simulink model "W07_alloc_chain"  (R2024b)
settings: Solver=ode4  StartTime=0  StopTime=T_final  FixedStep=h  RelTol=1e-3
InitFcn:
  | addpath(fullfile(fileparts(fileparts(fileparts(get_param(bdroot, 'FileName')))), '_tools'), fileparts(get_param(bdroot, 'FileName'))); run_alone('W07', bdroot);
StopFcn:
  | W07_plot_ca;
values from neighbouring files (symbols this model uses):
  alpha_lim = cfg.alpha_max(1)    [W07_0_setup.m]
  B_alloc = cfg.B    [W07_0_setup.m]
  beta_c = pi/2    (= 1.57079632679)    [W07_0_setup.m]
  eps_reg = 1e-4    (= 0.0001)    [W07_0_setup.m]    (also in W07_alloc_run.m)
  k_neg = cfg.k_neg    [W07_0_setup.m]
  k_pos = cfg.k_pos    [W07_0_setup.m]
  law = 4    [W07_0_setup.m]
  mp = 25    [W07_0_setup.m]
  n_max = cfg.n_max    [W07_0_setup.m]    (also in W07_plot_ca.m = base_num('n_max',      103.93); W07_plot_sat.m = base_var('n_max',      103.931))
  n_min = cfg.n_min    [W07_0_setup.m]    (also in W07_plot_ca.m = base_num('n_min',     -101.74); W07_plot_sat.m = base_var('n_min',     -101.737))
  Q_tau = eye(3)    [W07_0_setup.m]    (also in W07_alloc_run.m)
  quad = [cfg.pos ; cfg.alpha_max ; cfg.mount]    [W07_0_setup.m]
  rp = [0.05 0 -0.35]'    [W07_0_setup.m]
  T_neg = cfg.k_neg * cfg.n_min^2    [W07_0_setup.m]    (also in W07_plot_ca.m = base_num('T_neg',       66.708); W07_plot_sat.m = base_var('T_neg',        66.708))
  T_pos = cfg.k_pos * cfg.n_max^2    [W07_0_setup.m]    (also in W07_plot_ca.m = base_num('T_pos',      119.682); W07_plot_sat.m = base_var('T_pos',       119.682))
  tau_cmd = [0; 40; 0]    [W07_0_setup.m]
  V_c = 0.0    (= 0)    [W07_0_setup.m]
  W_alloc = diag(repmat([1 10], 1, 4))    [W07_0_setup.m]
  x0 = zeros(12,1)    [W07_0_setup.m]
settings Model: Creator=admin  LastModifiedBy=admin
settings DataIOCC: ReturnWorkspaceOutputs=off

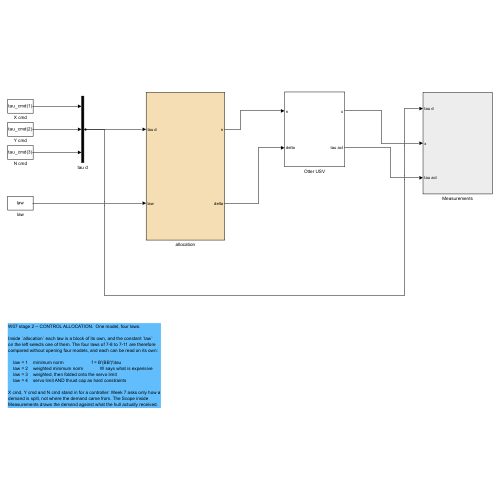
[thumbnail: Simulink's stored preview of the top-level diagram]
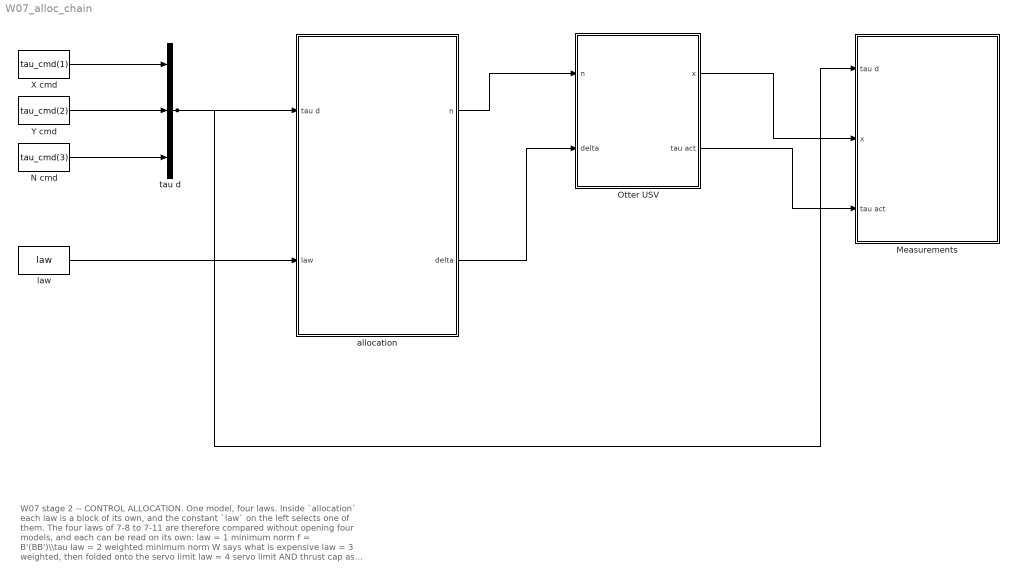
== system W07_alloc_chain ==
  note: W07 stage 2 -- CONTROL ALLOCATION.  One model, four laws.
      |
      | Inside `allocation` each law is a block of its own, and the constant `law`
      | on the left selects one of them. The four laws of 7-8 to 7-11 are therefore
      | compared without opening four models, and each can be read on its own:
      |
      |     law = 1    minimum norm                      f = B'(BB')\\tau
      |     law = 2    weighted minimum norm             W says what is expensive
      |     law = 3    weighted, then folded onto the servo limit
      |     law = 4    servo limit AND thrust cap as hard constraints
      |
      | X cmd, Y cmd and N cmd stand in for a controller: Week 7 asks only how a
      | demand is split, not where the demand came from. The Scope inside
      | Measurements draws the demand against what the hull actually received.
  Measurements : Subsystem
  N cmd : Constant  Value=tau_cmd(3)
  Otter USV : Subsystem
  X cmd : Constant  Value=tau_cmd(1)
  Y cmd : Constant  Value=tau_cmd(2)
  allocation : Subsystem
  law : Constant  Value=law
  tau d : Mux  Inputs=3
  wires:
  tau d/1 -> allocation/1(tau d), Measurements/1(tau d)
  law/1 -> allocation/2(law)
  X cmd/1 -> tau d/1
  Y cmd/1 -> tau d/2
  N cmd/1 -> tau d/3
  allocation/1(n) -> Otter USV/1(n)
  allocation/2(delta) -> Otter USV/2(delta)
  Otter USV/1(x) -> Measurements/2(x)
  Otter USV/2(tau act) -> Measurements/3(tau act)

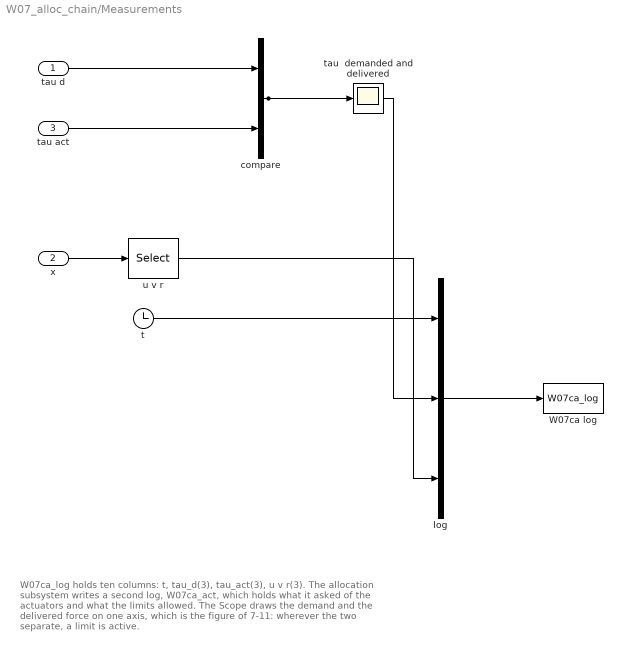
== system W07_alloc_chain/Measurements ==
  note: W07ca_log holds ten columns:  t,  tau_d(3),  tau_act(3),  u v r(3).
      | The allocation subsystem writes a second log, W07ca_act, which holds what
      | it asked of the actuators and what the limits allowed.
      |
      | The Scope draws the demand and the delivered force on one axis, which is
      | the figure of 7-11: wherever the two separate, a limit is active.
  tau d : Inport
  x : Inport  Port=2
  tau act : Inport  Port=3
  W07ca log : ToWorkspace  VariableName=W07ca_log  SampleTime=-1
  compare : Mux  Inputs=2
  log : Mux  Inputs=3
  t : Clock
  tau  demanded and delivered : Scope
  u v r : Selector  InputPortWidth=12  IndexOptions=Index vector (dialog)  Indices=[1 2 3]  OutputSizes=1
  wires:
  tau d/1 -> compare/1
  tau act/1 -> compare/2
  x/1 -> u v r/1
  t/1 -> log/1
  compare/1 -> tau  demanded and delivered/1, log/2
  log/1 -> W07ca log/1
  u v r/1 -> log/3

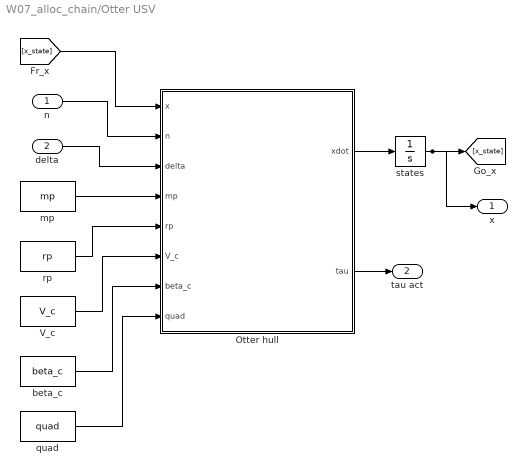
== system W07_alloc_chain/Otter USV ==
  n : Inport
  delta : Inport  Port=2
  Otter hull : MATLAB Function  TreatAsAtomicUnit=on
  V_c : Constant  Value=V_c
  beta_c : Constant  Value=beta_c
  mp : Constant  Value=mp
  quad : Constant  Value=quad
  rp : Constant  Value=rp
  states : Integrator  InitialCondition=x0
  x : Outport
  tau act : Outport  Port=2
  wires:
  rp/1 -> Otter hull/5(rp)
  delta/1 -> Otter hull/3(delta)
  [x_state] -> Otter hull/1(x)
  beta_c/1 -> Otter hull/7(beta_c)
  V_c/1 -> Otter hull/6(V_c)
  n/1 -> Otter hull/2(n)
  mp/1 -> Otter hull/4(mp)
  quad/1 -> Otter hull/8(quad)
  Otter hull/1(xdot) -> states/1
  states/1 -> [x_state], x/1
  Otter hull/2(tau) -> tau act/1

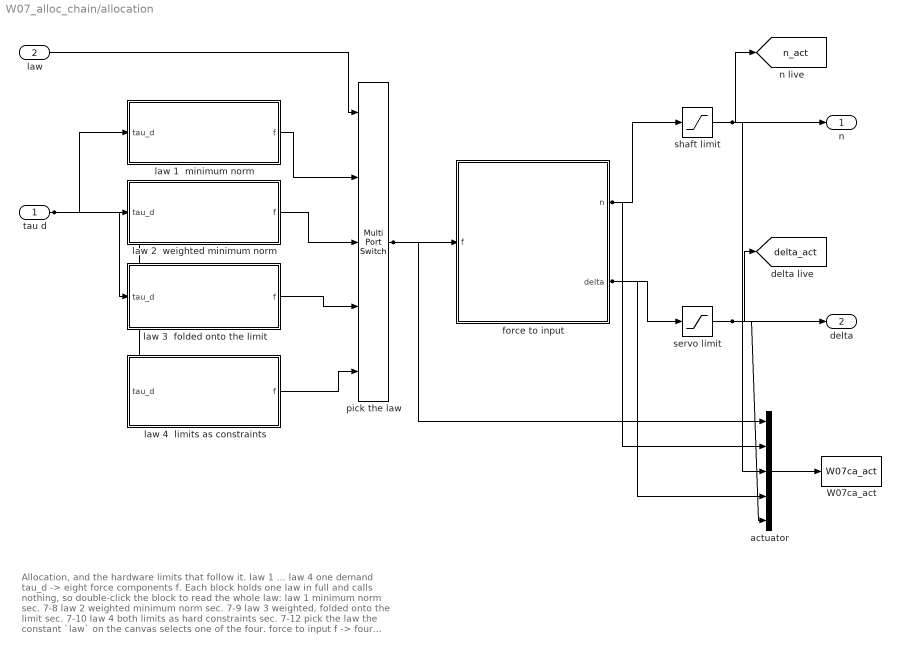
== system W07_alloc_chain/allocation ==
  note: Allocation, and the hardware limits that follow it.
      |
      | law 1 ... law 4   one demand tau_d -> eight force components f. Each block
      |                   holds one law in full and calls nothing, so double-click
      |                   the block to read the whole law:
      |
      |                       law 1   minimum norm                      sec. 7-8
      |                       law 2   weighted minimum norm             sec. 7-9
      |                       law 3   weighted, folded onto the limit   sec. 7-10
      |                       law 4   both limits as hard constraints   sec. 7-12
      |
      | pick the law      the constant `law` on the canvas selects one of the four.
      | force to input    f -> four shaft speeds n and four tilt angles delta. The
      |                   thrust sign is taken first, which is what folds every
      |                   angle into [-90, +90] deg before the servo ever sees it.
      |                   A unit asked for less than 0.5 N is held at n = 0 and
      |                   delta = 0, because below that the angle is arithmetic
      |                   noise and the servo would chatter at rest.
      | shaft limit       n clipped to [n_min, n_max].
      | servo limit       delta clipped to +-alpha_lim.
      | n live            the two clipped commands also leave as the global tags
      | delta live        n_act and delta_act, so the live view can draw them
      |                   against their limits while the run is still going. The
      |                   record below is readable only after it ends.
      | actuator          the record of this solve, written to W07ca_act as 24
      |                   columns:  f(8),  n asked(4),  n allowed(4),  delta
      |                   asked(4),  delta allowed(4). Wherever asked and allowed
      |                   differ, that unit is against a limit.
      |
      | What the hull was actually given is not rebuilt here: the motion model
      | already forms it from the clipped n and delta and reports it on its own
      | second output.
  tau d : Inport
  law : Inport  Port=2
  W07ca_act : ToWorkspace  VariableName=W07ca_act  SampleTime=-1
  actuator : Mux  Inputs=5
  force to input : MATLAB Function  TreatAsAtomicUnit=on
  law 1  minimum norm : MATLAB Function  TreatAsAtomicUnit=on
  law 2  weighted minimum norm : MATLAB Function  TreatAsAtomicUnit=on
  law 3  folded onto the limit : MATLAB Function  TreatAsAtomicUnit=on
  law 4  limits as constraints : MATLAB Function  TreatAsAtomicUnit=on
  pick the law : MultiPortSwitch  Inputs=4  SaturateOnIntegerOverflow=off  InputSameDT=off
  servo limit : Saturate  UpperLimit=alpha_lim  LowerLimit=-alpha_lim
  shaft limit : Saturate  UpperLimit=n_max  LowerLimit=n_min
  n : Outport
  delta : Outport  Port=2
  tag scope: delta_act=global, n_act=global
  wires:
  tau d/1 -> law 1  minimum norm/1(tau_d), law 2  weighted minimum norm/1(tau_d), law 3  folded onto the limit/1(tau_d), law 4  limits as constraints/1(tau_d)
  law/1 -> pick the law/1
  law 1  minimum norm/1(f) -> pick the law/2
  law 2  weighted minimum norm/1(f) -> pick the law/3
  law 3  folded onto the limit/1(f) -> pick the law/4
  law 4  limits as constraints/1(f) -> pick the law/5
  pick the law/1 -> force to input/1(f), actuator/1
  force to input/1(n) -> shaft limit/1, actuator/2
  force to input/2(delta) -> servo limit/1, actuator/4
  shaft limit/1 -> n/1, [n_act], actuator/3
  servo limit/1 -> delta/1, [delta_act], actuator/5
  actuator/1 -> W07ca_act/1

== matlab function W07_alloc_chain/allocation/law 2  weighted minimum norm ==
  data: tau_d input; f output double size=[8 1]; B_alloc parameter; W_alloc parameter
function f = law2_weighted_minimum_norm(tau_d, B_alloc, W_alloc)
% LAW 2 -- weighted minimum norm.  Section 7-9.
%
%     min f' W f    subject to    B f = tau_d
%     ->    f = W^-1 B' (B W^-1 B')^-1 tau_d
%
% W states what is expensive. With W = diag([1 10 1 10 ...]) the sway
% component of a unit costs ten times its surge component, so the solution
% leans on the shaft speeds rather than on the tilt angles.
Wi = W_alloc \ eye(8);
f  = Wi * B_alloc' * ((B_alloc*Wi*B_alloc') \ tau_d);
end

== matlab function W07_alloc_chain/allocation/law 1  minimum norm ==
  data: tau_d input; f output double size=[8 1]; B_alloc parameter
function f = law1_minimum_norm(tau_d, B_alloc)
% LAW 1 -- minimum norm.  Section 7-8.
%
%     min f'f    subject to    B f = tau_d       ->    f = B'(B B')\tau_d
%
% Eight unknowns against three equations: the demand leaves five directions
% free, and this law spends them on the shortest f. Nothing here knows about
% the servo limit or the thrust cap, which is what laws 3 and 4 go on to fix.
%
%     f = [f_x1; f_y1; f_x2; f_y2; f_x3; f_y3; f_x4; f_y4]
f = B_alloc' * ((B_alloc*B_alloc') \ tau_d);
end

== matlab function W07_alloc_chain/allocation/law 3  folded onto the limit ==
  data: tau_d input; f output double size=[8 1]; B_alloc parameter; W_alloc parameter; alpha_lim parameter
function f = law3_folded_onto_the_limit(tau_d, B_alloc, W_alloc, alpha_lim)
% LAW 3 -- the weighted solution, folded onto the servo limit.  Section 7-10.
%
% Law 2 can ask for a tilt angle no servo can reach. This law solves law 2
% first, then folds each angle back onto [-alpha_lim, +alpha_lim] while
% keeping the thrust magnitude of that unit:
%
%     T_i     = sigma_i |f_i|
%     delta_i = atan2(sigma_i f_yi, sigma_i f_xi)
%     delta_i <- min(max(delta_i, -alpha_lim), +alpha_lim)
%     f_i     <- T_i [cos delta_i ; sin delta_i]
%
% The fold treats each unit on its own, so the eight components no longer
% satisfy B f = tau_d. The error that opens up is the result of section 7-10.
Wi = W_alloc \ eye(8);
f  = Wi * B_alloc' * ((B_alloc*Wi*B_alloc') \ tau_d);

for i = 1:4
    fx = f(2*i-1);
    fy = f(2*i);
    s  = sign(fx);
    if s == 0
        s = 1;        % a unit with no surge component is left pointing abeam
    end
    T  = s * hypot(fx, fy);
    de = atan2(s*fy, s*fx);
    de = min(max(de, -alpha_lim), alpha_lim);
    f(2*i-1) = T * cos(de);
    f(2*i)   = T * sin(de);
end
end

== matlab function W07_alloc_chain/allocation/law 4  limits as constraints ==
  data: tau_d input; f output double size=[8 1]; B_alloc parameter; W_alloc parameter; alpha_lim parameter; Q_tau parameter; eps_reg parameter; T_pos parameter; T_neg parameter
function f = law4_limits_as_constraints(tau_d, B_alloc, W_alloc, alpha_lim, Q_tau, eps_reg, T_pos, T_neg)
% LAW 4 -- the servo limit AND the thrust cap as hard constraints.  7-12.
%
% Minimise   ||Q (B f - tau_d)||^2 + eps ||W^(1/2) f||^2
% subject to, for every unit i,
%
%     |f_yi| <= tan(alpha_lim) sigma_i f_xi               the servo limit
%     cos(th) x' + sin(th) y' <= R cos(alpha_lim/M)       the thrust cap
%
% written in unit axes x' = sigma_i f_xi and y' = sigma_i f_yi. Both are
% straight lines once the thrust sign sigma_i of that unit is fixed, so the
% problem is a QP: no local minima. The signs are not known in advance, so
% all 2^4 = 16 sign combinations are solved and the cheapest feasible one is
% kept. tau_d sits in the cost rather than in an equality, so a solution
% exists even when the demand cannot be delivered.
%
% The cap is an arc, which no QP can hold. It is replaced by M = 3 inscribed
% chords: neighbouring chords meet exactly on the circle of radius R and
% their midpoints sit at cos(15 deg) = 0.966 R, so the polygon never breaks
% the cap and is at worst 3.4 per cent conservative.
%
% lsqlin has no code generation support, so the call is extrinsic and every
% output it returns is given a size and a type beforehand.
coder.extrinsic('lsqlin', 'optimoptions');

M = 3;                   % chords per cone, the n_chord of W07_vars
t = tan(alpha_lim);

% the whole cost as one least-squares residual,  ||C f - d||
C = [Q_tau*B_alloc ; sqrt(eps_reg)*sqrt(W_alloc)];
d = [Q_tau*tau_d   ; zeros(8,1)];

% the fallback, used if no sign combination turns out to be feasible
Wi = W_alloc \ eye(8);
f  = Wi * B_alloc' * ((B_alloc*Wi*B_alloc') \ tau_d);

opts = optimoptions('lsqlin', 'Display', 'off');
best = inf;

for p = 0:15
    % the four thrust signs of combination p, read off its four bits
    sg = zeros(4,1);
    for i = 1:4
        sg(i) = 1 - 2*mod(floor(p/2^(i-1)), 2);
    end

    A = zeros(4*(2+M), 8);
    b = zeros(4*(2+M), 1);
    r = 0;
    for i = 1:4
        s = sg(i);
        if s > 0
            R = T_pos;
        else
            R = T_neg;    % written positive, so the cap is a radius
        end
        r = r + 1;  A(r, 2*i-1) = -t*s;  A(r, 2*i) =  1;
        r = r + 1;  A(r, 2*i-1) = -t*s;  A(r, 2*i) = -1;
        for j = 1:M
            th = -alpha_lim + (j - 0.5)*(2*alpha_lim/M);
            r  = r + 1;
            A(r, 2*i-1) = s*cos(th);
            A(r, 2*i)   = s*sin(th);
            b(r)        = R*cos(alpha_lim/M);
        end
    end

    x   = zeros(8,1);
    cst = 0;
    res = zeros(11,1);
    ef  = 0;
    [x, cst, res, ef] = lsqlin(C, d, A, b, [], [], [], [], [], opts);

    % a cost is a cost only where the solver reported a solution
    if ef > 0 && cst < best
        best = cst;
        f    = x;
    end
end
end

== matlab function W07_alloc_chain/allocation/force to input ==
  data: f input; n output double size=[4 1]; delta output; k_pos parameter; k_neg parameter
function [n, delta] = force2input(f, k_pos, k_neg)
% Eight force components -> four shaft speeds and four tilt angles.
%
%     sigma_i = sign(f_xi)                        which way the unit pushes
%     T_i     = sigma_i |f_i|                     signed thrust        [N]
%     delta_i = atan2(sigma_i f_yi, sigma_i f_xi) tilt angle         [rad]
%     n_i     = sign(T_i) sqrt(|T_i| / k_i)       shaft speed      [rad/s]
%
% Multiplying BOTH arguments of atan2 by sigma_i turns the direction through
% exactly pi, and because sigma_i f_xi >= 0 the result always lands in
% [-pi/2, +pi/2]. That is what keeps the angle reachable: a unit pushing
% astern comes out as negative thrust at a small angle instead of positive
% thrust at 180 deg, which no servo limited to +-45 deg could hold.
fx = f(1:2:7);
fy = f(2:2:8);
s  = sign(fx);
s(s == 0) = 1;      % a unit with no surge component is left pointing abeam

T     = s .* hypot(fx, fy);
delta = atan2(s.*fy, s.*fx);

% The coefficient depends on the sign because a propeller pushing astern is
% less efficient than the same propeller pushing ahead.
k = k_pos*double(T >= 0) + k_neg*double(T < 0);
n = sign(T) .* sqrt(abs(T) ./ k);

% Below a tiny force the angle stops meaning anything: atan2 of two numbers
% near zero turns with the last bit of the arithmetic, so a servo asked to
% follow it would chatter while the vessel sits still. Hold such a unit at
% zero instead. The threshold is 0.5 N, which is 0.4 % of the ahead cap, so
% no force a controller could usefully ask for is thrown away here.
tiny = hypot(fx, fy) < 0.5;
delta(tiny) = 0;
n(tiny)     = 0;
end

== matlab function W07_alloc_chain/Otter USV/Otter hull ==
  data: x input; xdot output double size=[12 1]; n input; delta input; mp input; rp input; V_c input; beta_c input; quad input; tau output double size=[3 1]
function [xdot, tau] = otter_hull(x, n, delta, mp, rp, V_c, beta_c, quad)
% otter_tilt4.m: Fossen's otter.m with four tilting thrusters, called
% unchanged from _tools. Four shaft speeds and four angles in, tau built
% inside, in the same four marked places as otter_bow.m.
%
%   x      12 states, fed back from the integrator
%   n      shaft speeds [rad/s], fore port / fore stbd / aft port / aft stbd
%   delta  tilt angles [rad], measured from the body x axis, CCW positive
%   quad   3 x 4: the x stations, the y stations and the tilt limits
%
% Rows 1, 2 and 6 of tau all carry the angles, by the column rule
% [e_x; e_y; x e_y - y e_x] with e = [cos delta; sin delta]. Nothing is
% added after the call; there is no superposition and no tau_ext port.
%
% The second output is the [X; Y; N] the model actually used, formed after n
% and delta are clipped to their limits. It is the delivered force, so no
% block outside has to rebuild it from n and delta.
%
% otter_tilt4.m is not written for code generation, so the call is extrinsic
% and both outputs have to be pre-sized for Simulink to know their widths.
coder.extrinsic('otter_tilt4');

xdot = zeros(12,1);
spd  = 0;
tau  = zeros(3,1);
[xdot, spd, tau] = otter_tilt4(x, n, delta, mp, rp, V_c, beta_c, quad);
end
